simulink model "Shaddad_System"  (R2026b)
undefined symbols (not defined in the file): P, scn_ic_elec_hw, Ts, VC_IMPL
libraries: simulink x4, sl3dlib x1
settings Model: Creator=aomar  LastModifiedBy=aomar

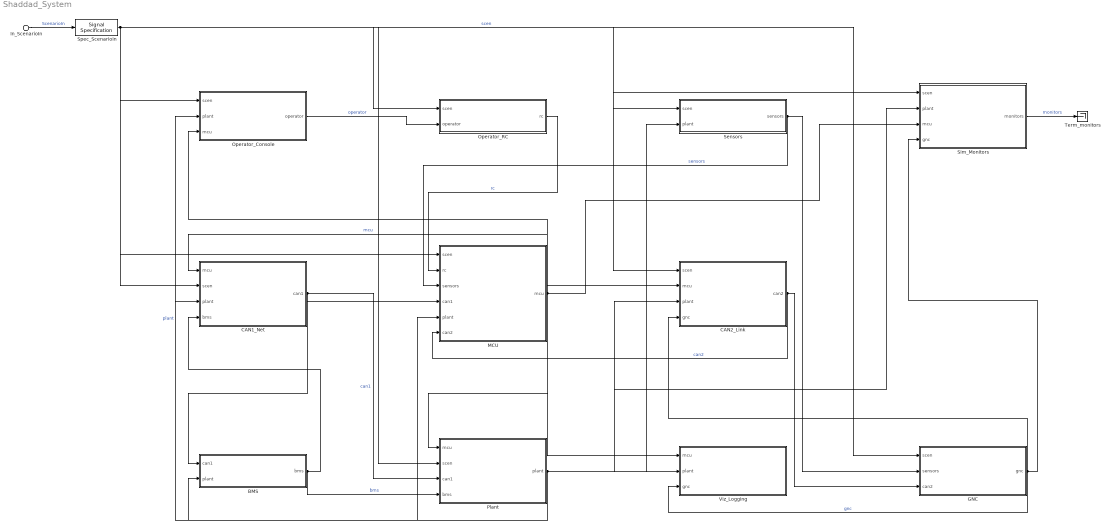
== system Shaddad_System ==
  In_ScenarioIn : Inport  PortName=ScenarioIn
  BMS : Subsystem  Description=BMS (ICD 3.1): Model Shaddad_BMS; its command leaves through BMS_Cmd_Delay (the ECU's one-sample compute delay, rule 8, D36) as bms.cmd_d.
  CAN1_Net : Subsystem
  CAN2_Link : Subsystem
  GNC : Subsystem  Description=GNC (ICD 3.1): MissionCmd_RT (0.01 -> 0.2 s, D32) and GNC_Variant (VC_PHASE 1 GNC_Stub, 2 Model Shaddad_Companion, D38).
  MCU : Subsystem  Description=MCU (ICD 3.1): MCU_In -> Model Shaddad_MCU. The CAN1 feedback frames and the ADC result reach the MCU one sample late (EscFb/EscSlow/Impl/Bms/Adc_Delay, rule 8, D36).
  Operator_Console : Subsystem  Description=VC_OPSRC 1 = ScenarioIn.op, 2 = dashboard (simulink_hmi_blocks bound to Constants, interactive runs), 3 = transmitter in USB joystick mode (Simulation 3D Joystick + joy_map, P.scen.joy), 4 = RC row test driver (row_driver_step, P.scen.rowdrv; fed the delayed true pose, speed, MCU mode and sprayer tank volume).
  Operator_RC : Subsystem
  Plant : Subsystem  Description=Plant (ICD 3.1): Model Shaddad_Plant; the DI word leaves through ElecHw_Delay (sampled by the MCU, rule 8, D36) as plant.elec_hw_d.
  Sensors : Subsystem
  Sim_Monitors : Subsystem
  Spec_ScenarioIn : SignalSpecification  OutDataTypeStr=Bus: Bus_ScenarioIn  SampleTime=Ts.scen  BusOutputAsStruct=on
  Term_monitors : Terminator
  Viz_Logging : Subsystem
  wires:
  In_ScenarioIn/1 -> Spec_ScenarioIn/1  "ScenarioIn"
  Spec_ScenarioIn/1 -> Plant/2(scen), GNC/1(scen), CAN1_Net/2(scen), CAN2_Link/1(scen), MCU/1(scen), Operator_RC/1(scen), Sensors/1(scen), Operator_Console/1(scen), Sim_Monitors/1(scen)  "scen"
  Operator_Console/1(operator) -> Operator_RC/2(operator)  "operator"
  CAN1_Net/1(can1) -> Plant/3(can1), BMS/1(can1), MCU/4(can1)  "can1"
  BMS/1(bms) -> CAN1_Net/4(bms), Plant/4(bms)  "bms"
  Operator_RC/1(rc) -> MCU/2(rc)  "rc"
  MCU/1(mcu) -> Sim_Monitors/3(mcu), Operator_Console/3(mcu), Viz_Logging/1(mcu), Plant/1(mcu), CAN1_Net/1(mcu), CAN2_Link/2(mcu)  "mcu"
  Plant/1(plant) -> Sim_Monitors/2(plant), Operator_Console/2(plant), Sensors/2(plant), CAN1_Net/3(plant), CAN2_Link/3(plant), MCU/5(plant), BMS/2(plant), Viz_Logging/2(plant)  "plant"
  Sensors/1(sensors) -> GNC/2(sensors), MCU/3(sensors)  "sensors"
  CAN2_Link/1(can2) -> GNC/3(can2), MCU/6(can2)  "can2"
  Sim_Monitors/1(monitors) -> Term_monitors/1  "monitors"
  GNC/1(gnc) -> Sim_Monitors/4(gnc), CAN2_Link/4(gnc), Viz_Logging/3(gnc)  "gnc"

== system Shaddad_System/BMS ==
  can1_mcu_slow_rx : Inport  PortName=can1  Element=mcu_slow_rx
  plant_bms_meas : Inport  Port=2  PortName=plant  Element=bms_meas
  BMS_Cmd_Delay : UnitDelay  InitialCondition=P.ic.Bus_BMS_Cmd  SampleTime=Ts.ctrl
  Shaddad_BMS : ModelReference  ModelNameDialog=Shaddad_BMS  SimulationMode=Normal  ModelReferenceVersion=1.1
  Spec_BMS_can_rx : SignalSpecification  OutDataTypeStr=Bus: Bus_Can1_McuSlow  SampleTime=Ts.comm  BusOutputAsStruct=on
  Spec_BMS_meas : SignalSpecification  OutDataTypeStr=Bus: Bus_BMS_Meas  SampleTime=Ts.ctrl  BusOutputAsStruct=on
  bms_cmd_d : Outport  PortName=bms  Element=cmd_d
  bms_can_tx : Outport  PortName=bms  Element=can_tx
  bms_telem : Outport  PortName=bms  Element=telem
  wires:
  plant_bms_meas/1 -> Spec_BMS_meas/1  "bms_meas"
  can1_mcu_slow_rx/1 -> Spec_BMS_can_rx/1  "mcu_slow_rx"
  Spec_BMS_meas/1 -> Shaddad_BMS/1  "meas"
  Spec_BMS_can_rx/1 -> Shaddad_BMS/2  "can_rx"
  Shaddad_BMS/1 -> BMS_Cmd_Delay/1  "cmd"
  Shaddad_BMS/2 -> bms_can_tx/1  "can_tx"
  Shaddad_BMS/3 -> bms_telem/1  "telem"
  BMS_Cmd_Delay/1 -> bms_cmd_d/1  "cmd_d"

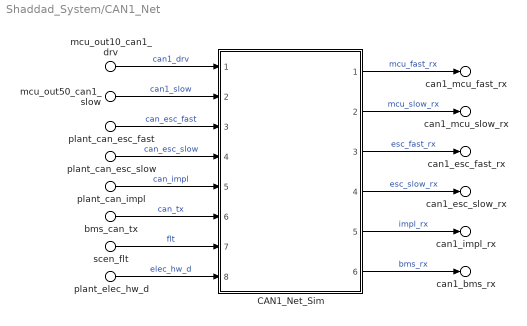
== system Shaddad_System/CAN1_Net ==
  mcu_out10_can1_drv : Inport  PortName=mcu  Element=out10.can1_drv
  mcu_out50_can1_slow : Inport  PortName=mcu  Element=out50.can1_slow
  scen_flt : Inport  Port=2  PortName=scen  Element=flt
  plant_can_esc_fast : Inport  Port=3  PortName=plant  Element=can_esc_fast
  plant_can_esc_slow : Inport  Port=3  PortName=plant  Element=can_esc_slow
  plant_can_impl : Inport  Port=3  PortName=plant  Element=can_impl
  plant_elec_hw_d : Inport  Port=3  PortName=plant  Element=elec_hw_d
  bms_can_tx : Inport  Port=4  PortName=bms  Element=can_tx
  CAN1_Net_Sim : Subsystem  ReferencedSubsystem=CAN1_Net_Sim
  can1_mcu_fast_rx : Outport  PortName=can1  Element=mcu_fast_rx
  can1_mcu_slow_rx : Outport  PortName=can1  Element=mcu_slow_rx
  can1_esc_fast_rx : Outport  PortName=can1  Element=esc_fast_rx
  can1_esc_slow_rx : Outport  PortName=can1  Element=esc_slow_rx
  can1_impl_rx : Outport  PortName=can1  Element=impl_rx
  can1_bms_rx : Outport  PortName=can1  Element=bms_rx
  wires:
  mcu_out10_can1_drv/1 -> CAN1_Net_Sim/1  "can1_drv"
  mcu_out50_can1_slow/1 -> CAN1_Net_Sim/2  "can1_slow"
  plant_can_esc_fast/1 -> CAN1_Net_Sim/3  "can_esc_fast"
  plant_can_esc_slow/1 -> CAN1_Net_Sim/4  "can_esc_slow"
  plant_can_impl/1 -> CAN1_Net_Sim/5  "can_impl"
  bms_can_tx/1 -> CAN1_Net_Sim/6  "can_tx"
  scen_flt/1 -> CAN1_Net_Sim/7  "flt"
  plant_elec_hw_d/1 -> CAN1_Net_Sim/8  "elec_hw_d"
  CAN1_Net_Sim/1 -> can1_mcu_fast_rx/1  "mcu_fast_rx"
  CAN1_Net_Sim/2 -> can1_mcu_slow_rx/1  "mcu_slow_rx"
  CAN1_Net_Sim/3 -> can1_esc_fast_rx/1  "esc_fast_rx"
  CAN1_Net_Sim/4 -> can1_esc_slow_rx/1  "esc_slow_rx"
  CAN1_Net_Sim/5 -> can1_impl_rx/1  "impl_rx"
  CAN1_Net_Sim/6 -> can1_bms_rx/1  "bms_rx"

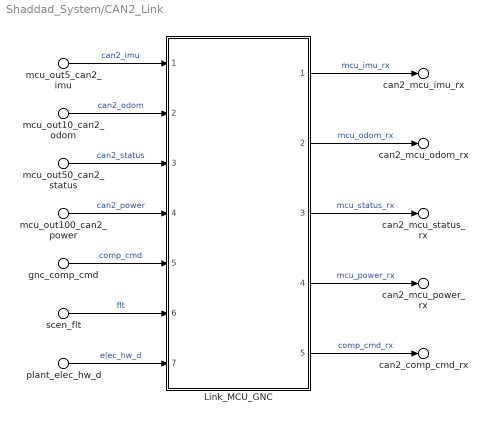
== system Shaddad_System/CAN2_Link ==
  scen_flt : Inport  PortName=scen  Element=flt
  mcu_out5_can2_imu : Inport  Port=2  PortName=mcu  Element=out5.can2_imu
  mcu_out10_can2_odom : Inport  Port=2  PortName=mcu  Element=out10.can2_odom
  mcu_out50_can2_status : Inport  Port=2  PortName=mcu  Element=out50.can2_status
  mcu_out100_can2_power : Inport  Port=2  PortName=mcu  Element=out100.can2_power
  plant_elec_hw_d : Inport  Port=3  PortName=plant  Element=elec_hw_d
  gnc_comp_cmd : Inport  Port=4  PortName=gnc  Element=comp_cmd
  Link_MCU_GNC : Subsystem  ReferencedSubsystem=Link_MCU_GNC
  can2_mcu_imu_rx : Outport  PortName=can2  Element=mcu_imu_rx
  can2_mcu_odom_rx : Outport  PortName=can2  Element=mcu_odom_rx
  can2_mcu_status_rx : Outport  PortName=can2  Element=mcu_status_rx
  can2_mcu_power_rx : Outport  PortName=can2  Element=mcu_power_rx
  can2_comp_cmd_rx : Outport  PortName=can2  Element=comp_cmd_rx
  wires:
  mcu_out5_can2_imu/1 -> Link_MCU_GNC/1  "can2_imu"
  mcu_out10_can2_odom/1 -> Link_MCU_GNC/2  "can2_odom"
  mcu_out50_can2_status/1 -> Link_MCU_GNC/3  "can2_status"
  mcu_out100_can2_power/1 -> Link_MCU_GNC/4  "can2_power"
  gnc_comp_cmd/1 -> Link_MCU_GNC/5  "comp_cmd"
  scen_flt/1 -> Link_MCU_GNC/6  "flt"
  plant_elec_hw_d/1 -> Link_MCU_GNC/7  "elec_hw_d"
  Link_MCU_GNC/1 -> can2_mcu_imu_rx/1  "mcu_imu_rx"
  Link_MCU_GNC/2 -> can2_mcu_odom_rx/1  "mcu_odom_rx"
  Link_MCU_GNC/3 -> can2_mcu_status_rx/1  "mcu_status_rx"
  Link_MCU_GNC/4 -> can2_mcu_power_rx/1  "mcu_power_rx"
  Link_MCU_GNC/5 -> can2_comp_cmd_rx/1  "comp_cmd_rx"

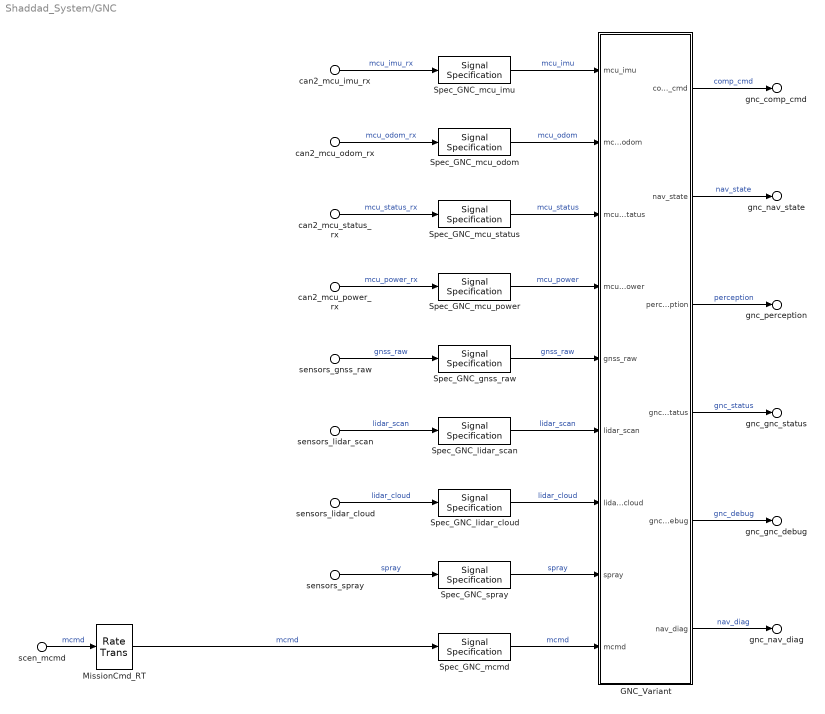
== system Shaddad_System/GNC ==
  scen_mcmd : Inport  PortName=scen  Element=mcmd
  sensors_gnss_raw : Inport  Port=2  PortName=sensors  Element=gnss_raw
  sensors_lidar_scan : Inport  Port=2  PortName=sensors  Element=lidar_scan
  sensors_lidar_cloud : Inport  Port=2  PortName=sensors  Element=lidar_cloud
  sensors_spray : Inport  Port=2  PortName=sensors  Element=spray
  can2_mcu_imu_rx : Inport  Port=3  PortName=can2  Element=mcu_imu_rx
  can2_mcu_odom_rx : Inport  Port=3  PortName=can2  Element=mcu_odom_rx
  can2_mcu_status_rx : Inport  Port=3  PortName=can2  Element=mcu_status_rx
  can2_mcu_power_rx : Inport  Port=3  PortName=can2  Element=mcu_power_rx
  GNC_Variant : Subsystem  Variant=on
  MissionCmd_RT : RateTransition  InitialCondition=P.ic.Bus_MissionCmd  OutPortSampleTime=Ts.mcmd
  Spec_GNC_gnss_raw : SignalSpecification  OutDataTypeStr=Bus: Bus_GnssRaw  SampleTime=Ts.hk  BusOutputAsStruct=on
  Spec_GNC_lidar_cloud : SignalSpecification  OutDataTypeStr=Bus: Bus_LidarCloudRaw  SampleTime=Ts.hk  BusOutputAsStruct=on
  Spec_GNC_lidar_scan : SignalSpecification  OutDataTypeStr=Bus: Bus_LidarScanRaw  SampleTime=Ts.hk  BusOutputAsStruct=on
  Spec_GNC_mcmd : SignalSpecification  OutDataTypeStr=Bus: Bus_MissionCmd  SampleTime=Ts.gnc_status  BusOutputAsStruct=on
  Spec_GNC_mcu_imu : SignalSpecification  OutDataTypeStr=Bus: Bus_CanFrame64  SampleTime=Ts.imu  BusOutputAsStruct=on
  Spec_GNC_mcu_odom : SignalSpecification  OutDataTypeStr=Bus: Bus_CanFrame64  SampleTime=Ts.ctrl  BusOutputAsStruct=on
  Spec_GNC_mcu_power : SignalSpecification  OutDataTypeStr=Bus: Bus_CanFrame64  SampleTime=Ts.hk  BusOutputAsStruct=on
  Spec_GNC_mcu_status : SignalSpecification  OutDataTypeStr=Bus: Bus_CanFrame64  SampleTime=Ts.comm  BusOutputAsStruct=on
  Spec_GNC_spray : SignalSpecification  OutDataTypeStr=Bus: Bus_SprayDemand  SampleTime=Ts.hk  BusOutputAsStruct=on
  gnc_comp_cmd : Outport  PortName=gnc  Element=comp_cmd
  gnc_nav_state : Outport  PortName=gnc  Element=nav_state
  gnc_perception : Outport  PortName=gnc  Element=perception
  gnc_gnc_status : Outport  PortName=gnc  Element=gnc_status
  gnc_gnc_debug : Outport  PortName=gnc  Element=gnc_debug
  gnc_nav_diag : Outport  PortName=gnc  Element=nav_diag
  wires:
  scen_mcmd/1 -> MissionCmd_RT/1  "mcmd"
  MissionCmd_RT/1 -> Spec_GNC_mcmd/1  "mcmd"
  can2_mcu_imu_rx/1 -> Spec_GNC_mcu_imu/1  "mcu_imu_rx"
  can2_mcu_odom_rx/1 -> Spec_GNC_mcu_odom/1  "mcu_odom_rx"
  can2_mcu_status_rx/1 -> Spec_GNC_mcu_status/1  "mcu_status_rx"
  can2_mcu_power_rx/1 -> Spec_GNC_mcu_power/1  "mcu_power_rx"
  sensors_gnss_raw/1 -> Spec_GNC_gnss_raw/1  "gnss_raw"
  sensors_lidar_scan/1 -> Spec_GNC_lidar_scan/1  "lidar_scan"
  sensors_lidar_cloud/1 -> Spec_GNC_lidar_cloud/1  "lidar_cloud"
  sensors_spray/1 -> Spec_GNC_spray/1  "spray"
  Spec_GNC_mcu_imu/1 -> GNC_Variant/1(mcu_imu)  "mcu_imu"
  Spec_GNC_mcu_odom/1 -> GNC_Variant/2(mcu_odom)  "mcu_odom"
  Spec_GNC_mcu_status/1 -> GNC_Variant/3(mcu_status)  "mcu_status"
  Spec_GNC_mcu_power/1 -> GNC_Variant/4(mcu_power)  "mcu_power"
  Spec_GNC_gnss_raw/1 -> GNC_Variant/5(gnss_raw)  "gnss_raw"
  Spec_GNC_lidar_scan/1 -> GNC_Variant/6(lidar_scan)  "lidar_scan"
  Spec_GNC_lidar_cloud/1 -> GNC_Variant/7(lidar_cloud)  "lidar_cloud"
  Spec_GNC_spray/1 -> GNC_Variant/8(spray)  "spray"
  Spec_GNC_mcmd/1 -> GNC_Variant/9(mcmd)  "mcmd"
  GNC_Variant/1(comp_cmd) -> gnc_comp_cmd/1  "comp_cmd"
  GNC_Variant/2(nav_state) -> gnc_nav_state/1  "nav_state"
  GNC_Variant/3(perception) -> gnc_perception/1  "perception"
  GNC_Variant/4(gnc_status) -> gnc_gnc_status/1  "gnc_status"
  GNC_Variant/5(gnc_debug) -> gnc_gnc_debug/1  "gnc_debug"
  GNC_Variant/6(nav_diag) -> gnc_nav_diag/1  "nav_diag"

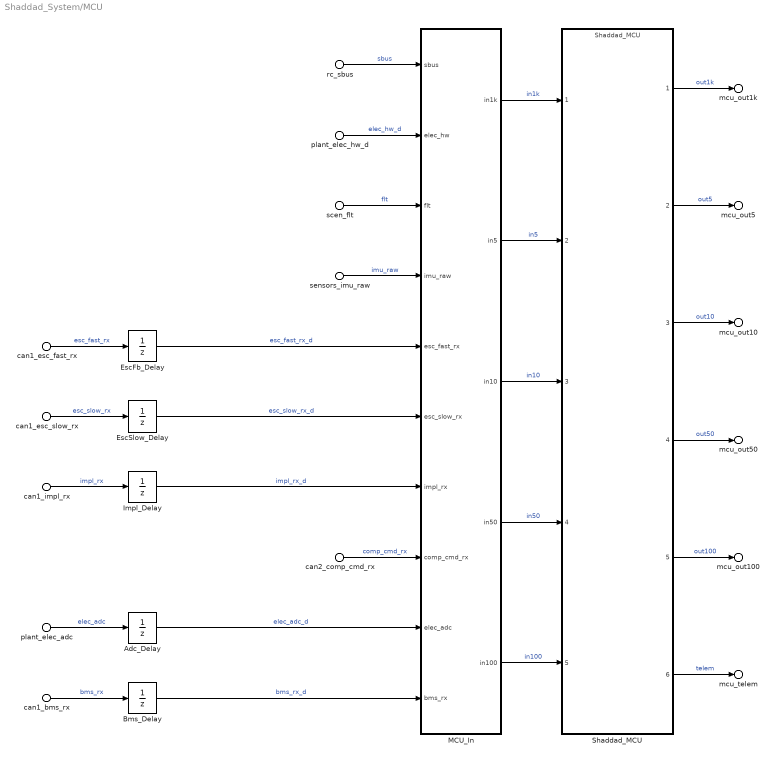
== system Shaddad_System/MCU ==
  scen_flt : Inport  PortName=scen  Element=flt
  rc_sbus : Inport  Port=2  PortName=rc  Element=sbus
  sensors_imu_raw : Inport  Port=3  PortName=sensors  Element=imu_raw
  can1_esc_fast_rx : Inport  Port=4  PortName=can1  Element=esc_fast_rx
  can1_esc_slow_rx : Inport  Port=4  PortName=can1  Element=esc_slow_rx
  can1_impl_rx : Inport  Port=4  PortName=can1  Element=impl_rx
  can1_bms_rx : Inport  Port=4  PortName=can1  Element=bms_rx
  plant_elec_hw_d : Inport  Port=5  PortName=plant  Element=elec_hw_d
  plant_elec_adc : Inport  Port=5  PortName=plant  Element=elec_adc
  can2_comp_cmd_rx : Inport  Port=6  PortName=can2  Element=comp_cmd_rx
  Adc_Delay : UnitDelay  InitialCondition=P.ic.Bus_ElecAdc  SampleTime=Ts.comm
  Bms_Delay : UnitDelay  InitialCondition=P.ic.Bus_Can1_Bms  SampleTime=Ts.hk
  EscFb_Delay : UnitDelay  InitialCondition=P.ic.Bus_Can1_EscFast  SampleTime=Ts.ctrl
  EscSlow_Delay : UnitDelay  InitialCondition=P.ic.Bus_Can1_EscSlow  SampleTime=Ts.comm
  Impl_Delay : UnitDelay  InitialCondition=P.ic.Bus_Can1_Impl  SampleTime=Ts.comm
  MCU_In : Subsystem  Description=MCU input assembly: explicit deterministic Rate Transitions to the task rates, nonvirtual Bus_McuIn* Bus Creators, t_us (1 MHz, wraps 2^32) and the SIM fault_inject word (ICD 6).
  Shaddad_MCU : ModelReference  ModelNameDialog=Shaddad_MCU  SimulationMode=Normal  ModelReferenceVersion=1.1
  mcu_out1k : Outport  PortName=mcu  Element=out1k
  mcu_out5 : Outport  PortName=mcu  Element=out5
  mcu_out10 : Outport  PortName=mcu  Element=out10
  mcu_out50 : Outport  PortName=mcu  Element=out50
  mcu_out100 : Outport  PortName=mcu  Element=out100
  mcu_telem : Outport  PortName=mcu  Element=telem
  wires:
  can1_esc_fast_rx/1 -> EscFb_Delay/1  "esc_fast_rx"
  can1_esc_slow_rx/1 -> EscSlow_Delay/1  "esc_slow_rx"
  can1_impl_rx/1 -> Impl_Delay/1  "impl_rx"
  plant_elec_adc/1 -> Adc_Delay/1  "elec_adc"
  can1_bms_rx/1 -> Bms_Delay/1  "bms_rx"
  EscFb_Delay/1 -> MCU_In/5(esc_fast_rx)  "esc_fast_rx_d"
  EscSlow_Delay/1 -> MCU_In/6(esc_slow_rx)  "esc_slow_rx_d"
  Impl_Delay/1 -> MCU_In/7(impl_rx)  "impl_rx_d"
  Adc_Delay/1 -> MCU_In/9(elec_adc)  "elec_adc_d"
  Bms_Delay/1 -> MCU_In/10(bms_rx)  "bms_rx_d"
  rc_sbus/1 -> MCU_In/1(sbus)  "sbus"
  plant_elec_hw_d/1 -> MCU_In/2(elec_hw)  "elec_hw_d"
  scen_flt/1 -> MCU_In/3(flt)  "flt"
  sensors_imu_raw/1 -> MCU_In/4(imu_raw)  "imu_raw"
  can2_comp_cmd_rx/1 -> MCU_In/8(comp_cmd_rx)  "comp_cmd_rx"
  MCU_In/1(in1k) -> Shaddad_MCU/1  "in1k"
  MCU_In/2(in5) -> Shaddad_MCU/2  "in5"
  MCU_In/3(in10) -> Shaddad_MCU/3  "in10"
  MCU_In/4(in50) -> Shaddad_MCU/4  "in50"
  MCU_In/5(in100) -> Shaddad_MCU/5  "in100"
  Shaddad_MCU/1 -> mcu_out1k/1  "out1k"
  Shaddad_MCU/2 -> mcu_out5/1  "out5"
  Shaddad_MCU/3 -> mcu_out10/1  "out10"
  Shaddad_MCU/4 -> mcu_out50/1  "out50"
  Shaddad_MCU/5 -> mcu_out100/1  "out100"
  Shaddad_MCU/6 -> mcu_telem/1  "telem"

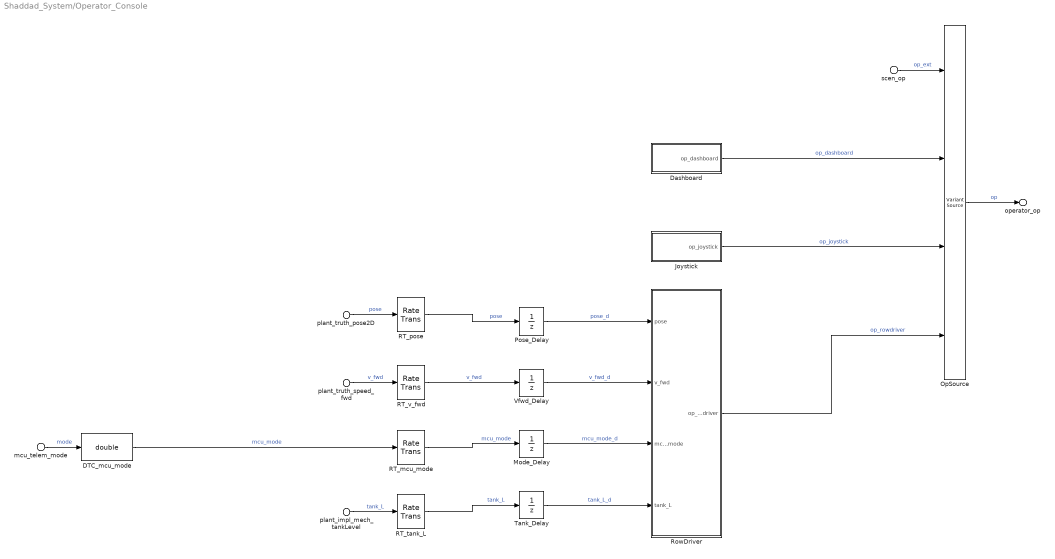
== system Shaddad_System/Operator_Console ==
  scen_op : Inport  PortName=scen  Element=op
  plant_truth_pose2D : Inport  Port=2  PortName=plant  Element=truth.pose2D
  plant_truth_speed_fwd : Inport  Port=2  PortName=plant  Element=truth.speed_fwd
  plant_impl_mech_tankLevel : Inport  Port=2  PortName=plant  Element=impl_mech.tankLevel
  mcu_telem_mode : Inport  Port=3  PortName=mcu  Element=telem.mode
  DTC_mcu_mode : DataTypeConversion  OutDataTypeStr=double  SaturateOnIntegerOverflow=off  RndMeth=Floor
  Dashboard : Subsystem  Description=VC_OPSRC 2: dashboard RC (simulink_hmi_blocks bound to the P.scen.dash Constants).
  Joystick : Subsystem  Description=VC_OPSRC 3: real transmitter in USB joystick mode (Simulation 3D Joystick, ID 1) mapped by utilities/joy_map.m with P.scen.joy; run phase1_live_drive('Source','joystick').
  Mode_Delay : UnitDelay  SampleTime=Ts.scen
  OpSource : VariantSource  VariantControls={VC_OPSRC == 1, VC_OPSRC == 2, VC_OPSRC == 3, VC_OPSRC == 4}
  Pose_Delay : UnitDelay  InitialCondition=P.structure.init.pose2D0  SampleTime=Ts.scen
  RT_mcu_mode : RateTransition  OutPortSampleTime=Ts.scen
  RT_pose : RateTransition  InitialCondition=P.structure.init.pose2D0  OutPortSampleTime=Ts.scen
  RT_tank_L : RateTransition  OutPortSampleTime=Ts.scen
  RT_v_fwd : RateTransition  OutPortSampleTime=Ts.scen
  RowDriver : Subsystem  Description=VC_OPSRC 4: RC row test driver (scenario R1, phase1_row_test): delayed true pose / speed, MCU mode and sprayer tank volume -> sticks and switches (the pump off once the tank is empty); Stop Simulation once the driver has ended the run.
  Tank_Delay : UnitDelay  SampleTime=Ts.scen
  Vfwd_Delay : UnitDelay  SampleTime=Ts.scen
  operator_op : Outport  PortName=operator  Element=op
  wires:
  mcu_telem_mode/1 -> DTC_mcu_mode/1  "mode"
  DTC_mcu_mode/1 -> RT_mcu_mode/1  "mcu_mode"
  plant_truth_pose2D/1 -> RT_pose/1  "pose"
  plant_truth_speed_fwd/1 -> RT_v_fwd/1  "v_fwd"
  plant_impl_mech_tankLevel/1 -> RT_tank_L/1  "tank_L"
  RT_pose/1 -> Pose_Delay/1  "pose"
  RT_v_fwd/1 -> Vfwd_Delay/1  "v_fwd"
  RT_mcu_mode/1 -> Mode_Delay/1  "mcu_mode"
  RT_tank_L/1 -> Tank_Delay/1  "tank_L"
  Pose_Delay/1 -> RowDriver/1(pose)  "pose_d"
  Vfwd_Delay/1 -> RowDriver/2(v_fwd)  "v_fwd_d"
  Mode_Delay/1 -> RowDriver/3(mcu_mode)  "mcu_mode_d"
  Tank_Delay/1 -> RowDriver/4(tank_L)  "tank_L_d"
  Dashboard/1(op_dashboard) -> OpSource/2  "op_dashboard"
  Joystick/1(op_joystick) -> OpSource/3  "op_joystick"
  RowDriver/1(op_rowdriver) -> OpSource/4  "op_rowdriver"
  scen_op/1 -> OpSource/1  "op_ext"
  OpSource/1 -> operator_op/1  "op"

== system Shaddad_System/Operator_RC ==
  scen_flt : Inport  PortName=scen  Element=flt
  operator_op : Inport  Port=2  PortName=operator  Element=op
  RC_Link_Sim : Subsystem  ReferencedSubsystem=RC_Link_Sim
  rc_sbus : Outport  PortName=rc  Element=sbus
  rc_rc_frame : Outport  PortName=rc  Element=rc_frame
  wires:
  operator_op/1 -> RC_Link_Sim/1  "op"
  scen_flt/1 -> RC_Link_Sim/2  "flt"
  RC_Link_Sim/1 -> rc_sbus/1  "sbus"
  RC_Link_Sim/2 -> rc_rc_frame/1  "rc_frame"

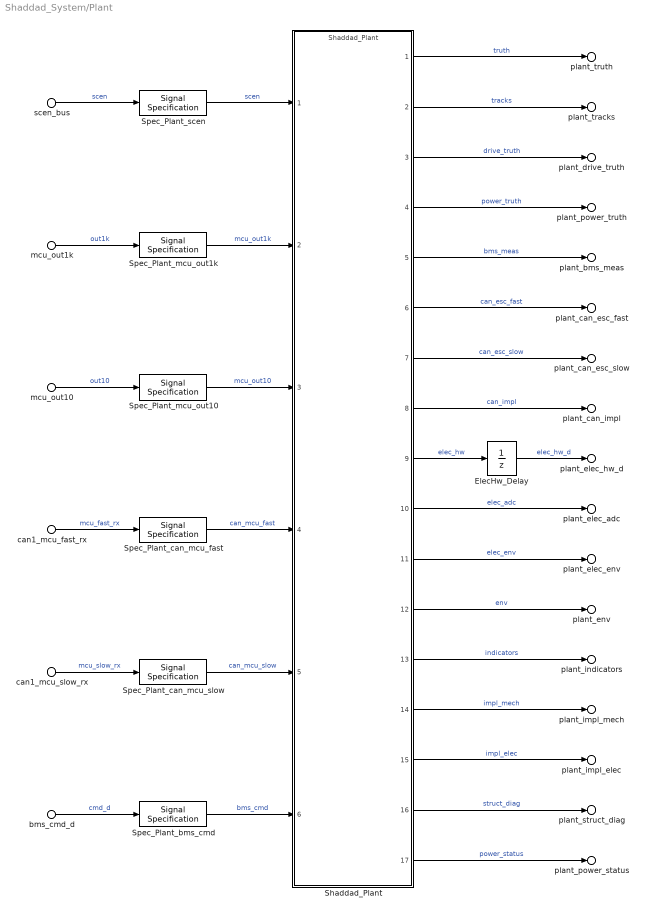
== system Shaddad_System/Plant ==
  mcu_out1k : Inport  PortName=mcu  Element=out1k
  mcu_out10 : Inport  PortName=mcu  Element=out10
  scen_bus : Inport  Port=2  PortName=scen
  can1_mcu_fast_rx : Inport  Port=3  PortName=can1  Element=mcu_fast_rx
  can1_mcu_slow_rx : Inport  Port=3  PortName=can1  Element=mcu_slow_rx
  bms_cmd_d : Inport  Port=4  PortName=bms  Element=cmd_d
  ElecHw_Delay : UnitDelay  InitialCondition=scn_ic_elec_hw(P, VC_IMPL)  SampleTime=Ts.base
  Shaddad_Plant : ModelReference  ModelNameDialog=Shaddad_Plant  SimulationMode=Normal  ModelReferenceVersion=1.1
  Spec_Plant_bms_cmd : SignalSpecification  OutDataTypeStr=Bus: Bus_BMS_Cmd  SampleTime=Ts.ctrl  BusOutputAsStruct=on
  Spec_Plant_can_mcu_fast : SignalSpecification  OutDataTypeStr=Bus: Bus_Can1_McuFast  SampleTime=Ts.ctrl  BusOutputAsStruct=on
  Spec_Plant_can_mcu_slow : SignalSpecification  OutDataTypeStr=Bus: Bus_Can1_McuSlow  SampleTime=Ts.comm  BusOutputAsStruct=on
  Spec_Plant_mcu_out10 : SignalSpecification  OutDataTypeStr=Bus: Bus_McuOut10  SampleTime=Ts.ctrl  BusOutputAsStruct=on
  Spec_Plant_mcu_out1k : SignalSpecification  OutDataTypeStr=Bus: Bus_McuOut1k  SampleTime=Ts.base  BusOutputAsStruct=on
  Spec_Plant_scen : SignalSpecification  OutDataTypeStr=Bus: Bus_ScenarioIn  SampleTime=Ts.ctrl  BusOutputAsStruct=on
  plant_truth : Outport  PortName=plant  Element=truth
  plant_tracks : Outport  PortName=plant  Element=tracks
  plant_drive_truth : Outport  PortName=plant  Element=drive_truth
  plant_power_truth : Outport  PortName=plant  Element=power_truth
  plant_bms_meas : Outport  PortName=plant  Element=bms_meas
  plant_can_esc_fast : Outport  PortName=plant  Element=can_esc_fast
  plant_can_esc_slow : Outport  PortName=plant  Element=can_esc_slow
  plant_can_impl : Outport  PortName=plant  Element=can_impl
  plant_elec_hw_d : Outport  PortName=plant  Element=elec_hw_d
  plant_elec_adc : Outport  PortName=plant  Element=elec_adc
  plant_elec_env : Outport  PortName=plant  Element=elec_env
  plant_env : Outport  PortName=plant  Element=env
  plant_indicators : Outport  PortName=plant  Element=indicators
  plant_impl_mech : Outport  PortName=plant  Element=impl_mech
  plant_impl_elec : Outport  PortName=plant  Element=impl_elec
  plant_struct_diag : Outport  PortName=plant  Element=struct_diag
  plant_power_status : Outport  PortName=plant  Element=power_status
  wires:
  scen_bus/1 -> Spec_Plant_scen/1  "scen"
  mcu_out1k/1 -> Spec_Plant_mcu_out1k/1  "out1k"
  mcu_out10/1 -> Spec_Plant_mcu_out10/1  "out10"
  can1_mcu_fast_rx/1 -> Spec_Plant_can_mcu_fast/1  "mcu_fast_rx"
  can1_mcu_slow_rx/1 -> Spec_Plant_can_mcu_slow/1  "mcu_slow_rx"
  bms_cmd_d/1 -> Spec_Plant_bms_cmd/1  "cmd_d"
  Spec_Plant_scen/1 -> Shaddad_Plant/1  "scen"
  Spec_Plant_mcu_out1k/1 -> Shaddad_Plant/2  "mcu_out1k"
  Spec_Plant_mcu_out10/1 -> Shaddad_Plant/3  "mcu_out10"
  Spec_Plant_can_mcu_fast/1 -> Shaddad_Plant/4  "can_mcu_fast"
  Spec_Plant_can_mcu_slow/1 -> Shaddad_Plant/5  "can_mcu_slow"
  Spec_Plant_bms_cmd/1 -> Shaddad_Plant/6  "bms_cmd"
  Shaddad_Plant/1 -> plant_truth/1  "truth"
  Shaddad_Plant/2 -> plant_tracks/1  "tracks"
  Shaddad_Plant/3 -> plant_drive_truth/1  "drive_truth"
  Shaddad_Plant/4 -> plant_power_truth/1  "power_truth"
  Shaddad_Plant/5 -> plant_bms_meas/1  "bms_meas"
  Shaddad_Plant/6 -> plant_can_esc_fast/1  "can_esc_fast"
  Shaddad_Plant/7 -> plant_can_esc_slow/1  "can_esc_slow"
  Shaddad_Plant/8 -> plant_can_impl/1  "can_impl"
  Shaddad_Plant/9 -> ElecHw_Delay/1  "elec_hw"
  Shaddad_Plant/10 -> plant_elec_adc/1  "elec_adc"
  Shaddad_Plant/11 -> plant_elec_env/1  "elec_env"
  Shaddad_Plant/12 -> plant_env/1  "env"
  Shaddad_Plant/13 -> plant_indicators/1  "indicators"
  Shaddad_Plant/14 -> plant_impl_mech/1  "impl_mech"
  Shaddad_Plant/15 -> plant_impl_elec/1  "impl_elec"
  Shaddad_Plant/16 -> plant_struct_diag/1  "struct_diag"
  Shaddad_Plant/17 -> plant_power_status/1  "power_status"
  ElecHw_Delay/1 -> plant_elec_hw_d/1  "elec_hw_d"

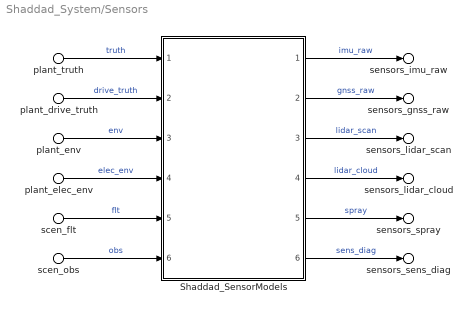
== system Shaddad_System/Sensors ==
  scen_flt : Inport  PortName=scen  Element=flt
  scen_obs : Inport  PortName=scen  Element=obs
  plant_truth : Inport  Port=2  PortName=plant  Element=truth
  plant_drive_truth : Inport  Port=2  PortName=plant  Element=drive_truth
  plant_env : Inport  Port=2  PortName=plant  Element=env
  plant_elec_env : Inport  Port=2  PortName=plant  Element=elec_env
  Shaddad_SensorModels : Subsystem  ReferencedSubsystem=Shaddad_SensorModels
  sensors_imu_raw : Outport  PortName=sensors  Element=imu_raw
  sensors_gnss_raw : Outport  PortName=sensors  Element=gnss_raw
  sensors_lidar_scan : Outport  PortName=sensors  Element=lidar_scan
  sensors_lidar_cloud : Outport  PortName=sensors  Element=lidar_cloud
  sensors_spray : Outport  PortName=sensors  Element=spray
  sensors_sens_diag : Outport  PortName=sensors  Element=sens_diag
  wires:
  plant_truth/1 -> Shaddad_SensorModels/1  "truth"
  plant_drive_truth/1 -> Shaddad_SensorModels/2  "drive_truth"
  plant_env/1 -> Shaddad_SensorModels/3  "env"
  plant_elec_env/1 -> Shaddad_SensorModels/4  "elec_env"
  scen_flt/1 -> Shaddad_SensorModels/5  "flt"
  scen_obs/1 -> Shaddad_SensorModels/6  "obs"
  Shaddad_SensorModels/1 -> sensors_imu_raw/1  "imu_raw"
  Shaddad_SensorModels/2 -> sensors_gnss_raw/1  "gnss_raw"
  Shaddad_SensorModels/3 -> sensors_lidar_scan/1  "lidar_scan"
  Shaddad_SensorModels/4 -> sensors_lidar_cloud/1  "lidar_cloud"
  Shaddad_SensorModels/5 -> sensors_spray/1  "spray"
  Shaddad_SensorModels/6 -> sensors_sens_diag/1  "sens_diag"

== system Shaddad_System/Sim_Monitors ==
  scen_obs : Inport  PortName=scen  Element=obs
  plant_truth : Inport  Port=2  PortName=plant  Element=truth
  plant_power_truth : Inport  Port=2  PortName=plant  Element=power_truth
  plant_drive_truth : Inport  Port=2  PortName=plant  Element=drive_truth
  plant_struct_diag : Inport  Port=2  PortName=plant  Element=struct_diag
  mcu_telem : Inport  Port=3  PortName=mcu  Element=telem
  gnc_gnc_status : Inport  Port=4  PortName=gnc  Element=gnc_status
  Sim_Monitors : Subsystem  ReferencedSubsystem=Sim_Monitors
  monitors_kpi : Outport  PortName=monitors  Element=kpi
  wires:
  plant_truth/1 -> Sim_Monitors/1  "truth"
  plant_power_truth/1 -> Sim_Monitors/2  "power_truth"
  plant_drive_truth/1 -> Sim_Monitors/3  "drive_truth"
  scen_obs/1 -> Sim_Monitors/4  "obs"
  mcu_telem/1 -> Sim_Monitors/5  "telem"
  gnc_gnc_status/1 -> Sim_Monitors/6  "gnc_status"
  plant_struct_diag/1 -> Sim_Monitors/7  "struct_diag"
  Sim_Monitors/1 -> monitors_kpi/1  "kpi"

== system Shaddad_System/Viz_Logging ==
  mcu_telem : Inport  PortName=mcu  Element=telem
  plant_truth : Inport  Port=2  PortName=plant  Element=truth
  plant_indicators : Inport  Port=2  PortName=plant  Element=indicators
  gnc_nav_state : Inport  Port=3  PortName=gnc  Element=nav_state
  gnc_gnc_status : Inport  Port=3  PortName=gnc  Element=gnc_status
  gnc_perception : Inport  Port=3  PortName=gnc  Element=perception
  Viz_Logging : Subsystem  ReferencedSubsystem=Viz_Logging
  wires:
  plant_truth/1 -> Viz_Logging/1  "truth"
  gnc_nav_state/1 -> Viz_Logging/2  "nav_state"
  gnc_gnc_status/1 -> Viz_Logging/3  "gnc_status"
  gnc_perception/1 -> Viz_Logging/4  "perception"
  mcu_telem/1 -> Viz_Logging/5  "telem"
  plant_indicators/1 -> Viz_Logging/6  "indicators"

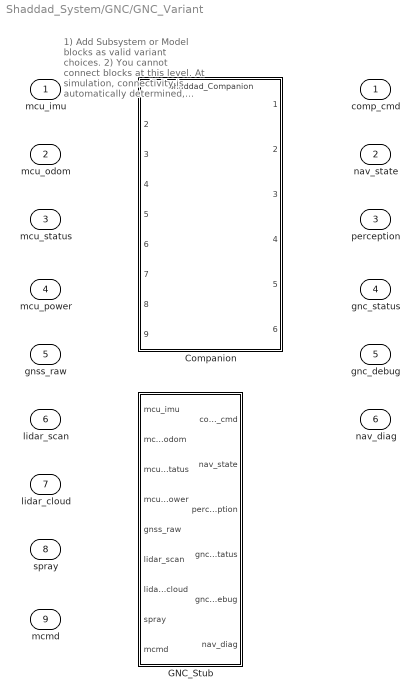
== system Shaddad_System/GNC/GNC_Variant ==
  note: 1) Add Subsystem or Model blocks as valid variant choices.
      | 2) You cannot connect blocks at this level. At simulation, connectivity is automatically
      | determined, based on the active variant and port name matching.
  mcu_imu : Inport
  mcu_odom : Inport  Port=2
  mcu_status : Inport  Port=3
  mcu_power : Inport  Port=4
  gnss_raw : Inport  Port=5
  lidar_scan : Inport  Port=6
  lidar_cloud : Inport  Port=7
  spray : Inport  Port=8
  mcmd : Inport  Port=9
  Companion : ModelReference  ModelNameDialog=Shaddad_Companion  SimulationMode=Normal  VariantControl=VC_PHASE == 2  ModelReferenceVersion=1.1
  GNC_Stub : Subsystem  Description=Phase 1 (RC only): no companion; COMP_CMD valid = false so the MCU never sees comp_ok.  VariantControl=VC_PHASE == 1
  comp_cmd : Outport
  nav_state : Outport  Port=2
  perception : Outport  Port=3
  gnc_status : Outport  Port=4
  gnc_debug : Outport  Port=5
  nav_diag : Outport  Port=6

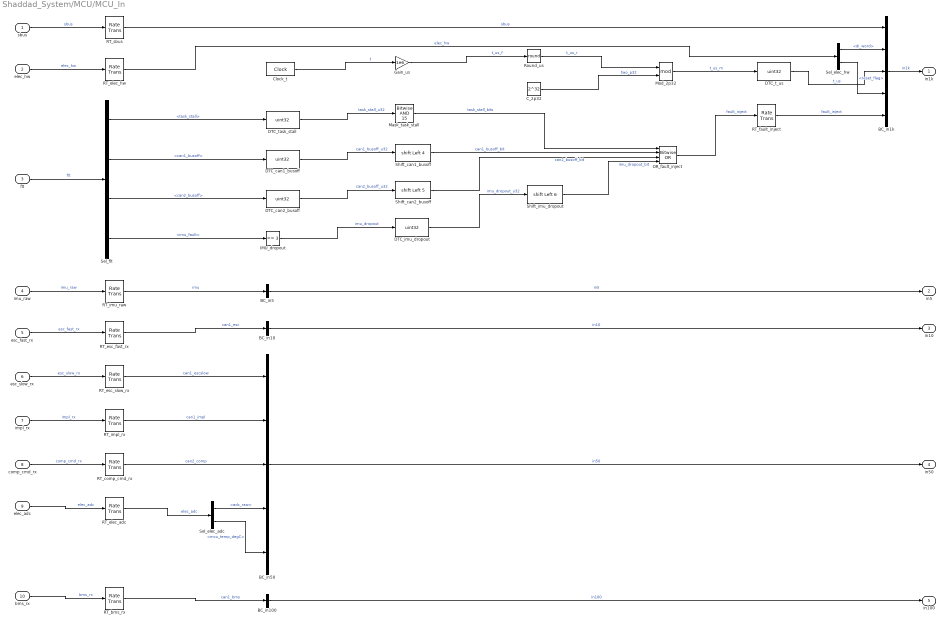
== system Shaddad_System/MCU/MCU_In ==
  sbus : Inport  OutDataTypeStr=Bus: Bus_SbusStream
  elec_hw : Inport  Port=2  OutDataTypeStr=Bus: Bus_ElecHwIn
  flt : Inport  Port=3  OutDataTypeStr=Bus: Bus_FaultInject
  imu_raw : Inport  Port=4  OutDataTypeStr=Bus: Bus_ImuRaw
  esc_fast_rx : Inport  Port=5  OutDataTypeStr=Bus: Bus_Can1_EscFast
  esc_slow_rx : Inport  Port=6  OutDataTypeStr=Bus: Bus_Can1_EscSlow
  impl_rx : Inport  Port=7  OutDataTypeStr=Bus: Bus_Can1_Impl
  comp_cmd_rx : Inport  Port=8  OutDataTypeStr=Bus: Bus_CanFrame64
  elec_adc : Inport  Port=9  OutDataTypeStr=Bus: Bus_ElecAdc
  bms_rx : Inport  Port=10  OutDataTypeStr=Bus: Bus_Can1_Bms
  BC_in10 : BusCreator  Inputs=1  OutDataTypeStr=Bus: Bus_McuIn10  NonVirtualBus=on
  BC_in100 : BusCreator  Inputs=1  OutDataTypeStr=Bus: Bus_McuIn100  NonVirtualBus=on
  BC_in1k : BusCreator  Inputs=5  OutDataTypeStr=Bus: Bus_McuIn1k  NonVirtualBus=on
  BC_in5 : BusCreator  Inputs=1  OutDataTypeStr=Bus: Bus_McuIn5  NonVirtualBus=on
  BC_in50 : BusCreator  Inputs=5  OutDataTypeStr=Bus: Bus_McuIn50  NonVirtualBus=on
  C_2p32 : Constant  Value=2^32
  Clock_t : DigitalClock  SampleTime=Ts.base
  DTC_can1_busoff : DataTypeConversion  OutDataTypeStr=uint32  SaturateOnIntegerOverflow=off  RndMeth=Floor
  DTC_can2_busoff : DataTypeConversion  OutDataTypeStr=uint32  SaturateOnIntegerOverflow=off  RndMeth=Floor
  DTC_imu_dropout : DataTypeConversion  OutDataTypeStr=uint32  SaturateOnIntegerOverflow=off  RndMeth=Floor
  DTC_t_us : DataTypeConversion  OutDataTypeStr=uint32  SaturateOnIntegerOverflow=off  RndMeth=Floor
  DTC_task_stall : DataTypeConversion  OutDataTypeStr=uint32  SaturateOnIntegerOverflow=off  RndMeth=Floor
  Gain_us : Gain  Gain=1e6
  IMU_dropout : simulink/Logic and Bit Operations/Compare To Constant  relop===  const=3  OutDataTypeStr=boolean
  Mask_task_stall : simulink/Logic and Bit Operations/Bitwise Operator  logicop=AND  UseBitMask=on  BitMask=15  BitMaskRealWorld=Stored Integer
  Mod_2p32 : Math  Operator=mod
  OR_fault_inject : simulink/Logic and Bit Operations/Bitwise Operator  logicop=OR  UseBitMask=off  NumInputPorts=4  BitMask=bin2dec('11011001')  BitMaskRealWorld=Stored Integer
  RT_bms_rx : RateTransition  InitialCondition=P.ic.Bus_Can1_Bms  OutPortSampleTime=Ts.hk
  RT_comp_cmd_rx : RateTransition  InitialCondition=P.ic.Bus_CanFrame64  OutPortSampleTime=Ts.comm
  RT_elec_adc : RateTransition  InitialCondition=P.ic.Bus_ElecAdc  OutPortSampleTime=Ts.comm
  RT_elec_hw : RateTransition  InitialCondition=P.ic.Bus_ElecHwIn  OutPortSampleTime=Ts.base
  RT_esc_fast_rx : RateTransition  InitialCondition=P.ic.Bus_Can1_EscFast  OutPortSampleTime=Ts.ctrl
  RT_esc_slow_rx : RateTransition  InitialCondition=P.ic.Bus_Can1_EscSlow  OutPortSampleTime=Ts.comm
  RT_fault_inject : RateTransition  OutPortSampleTime=Ts.base
  RT_impl_rx : RateTransition  InitialCondition=P.ic.Bus_Can1_Impl  OutPortSampleTime=Ts.comm
  RT_imu_raw : RateTransition  InitialCondition=P.ic.Bus_ImuRaw  OutPortSampleTime=Ts.imu
  RT_sbus : RateTransition  InitialCondition=P.ic.Bus_SbusStream  OutPortSampleTime=Ts.base
  Round_us : Rounding  Operator=round
  Sel_elec_adc : BusSelector  OutputSignals=adc_raw,mcu_temp_degC
  Sel_elec_hw : BusSelector  OutputSignals=di_word,reset_flag
  Sel_flt : BusSelector  OutputSignals=task_stall,can1_busoff,can2_busoff,imu_fault
  Shift_can1_busoff : ArithShift  BitShiftNumber=4  BitShiftDirection=Left
  Shift_can2_busoff : ArithShift  BitShiftNumber=5  BitShiftDirection=Left
  Shift_imu_dropout : ArithShift  BitShiftNumber=6  BitShiftDirection=Left
  in1k : Outport  OutDataTypeStr=Bus: Bus_McuIn1k
  in5 : Outport  Port=2  OutDataTypeStr=Bus: Bus_McuIn5
  in10 : Outport  Port=3  OutDataTypeStr=Bus: Bus_McuIn10
  in50 : Outport  Port=4  OutDataTypeStr=Bus: Bus_McuIn50
  in100 : Outport  Port=5  OutDataTypeStr=Bus: Bus_McuIn100
  wires:
  sbus/1 -> RT_sbus/1  "sbus"
  elec_hw/1 -> RT_elec_hw/1  "elec_hw"
  flt/1 -> Sel_flt/1  "flt"
  imu_raw/1 -> RT_imu_raw/1  "imu_raw"
  esc_fast_rx/1 -> RT_esc_fast_rx/1  "esc_fast_rx"
  esc_slow_rx/1 -> RT_esc_slow_rx/1  "esc_slow_rx"
  impl_rx/1 -> RT_impl_rx/1  "impl_rx"
  comp_cmd_rx/1 -> RT_comp_cmd_rx/1  "comp_cmd_rx"
  elec_adc/1 -> RT_elec_adc/1  "elec_adc"
  bms_rx/1 -> RT_bms_rx/1  "bms_rx"
  Sel_flt/1 -> DTC_task_stall/1  "<task_stall>"
  Sel_flt/2 -> DTC_can1_busoff/1  "<can1_busoff>"
  Sel_flt/3 -> DTC_can2_busoff/1  "<can2_busoff>"
  Sel_flt/4 -> IMU_dropout/1  "<imu_fault>"
  RT_sbus/1 -> BC_in1k/1  "sbus"
  RT_elec_hw/1 -> Sel_elec_hw/1  "elec_hw"
  RT_imu_raw/1 -> BC_in5/1  "imu"
  RT_esc_fast_rx/1 -> BC_in10/1  "can1_esc"
  RT_esc_slow_rx/1 -> BC_in50/1  "can1_escslow"
  RT_impl_rx/1 -> BC_in50/2  "can1_impl"
  RT_comp_cmd_rx/1 -> BC_in50/3  "can2_comp"
  RT_elec_adc/1 -> Sel_elec_adc/1  "elec_adc"
  RT_bms_rx/1 -> BC_in100/1  "can1_bms"
  Sel_elec_adc/1 -> BC_in50/4  "<adc_raw>"
  Sel_elec_adc/2 -> BC_in50/5  "<mcu_temp_degC>"
  BC_in5/1 -> in5/1  "in5"
  BC_in10/1 -> in10/1  "in10"
  BC_in50/1 -> in50/1  "in50"
  BC_in100/1 -> in100/1  "in100"
  IMU_dropout/1 -> DTC_imu_dropout/1  "imu_dropout"
  Clock_t/1 -> Gain_us/1  "t"
  DTC_task_stall/1 -> Mask_task_stall/1  "task_stall_u32"
  DTC_can1_busoff/1 -> Shift_can1_busoff/1  "can1_busoff_u32"
  DTC_can2_busoff/1 -> Shift_can2_busoff/1  "can2_busoff_u32"
  Gain_us/1 -> Round_us/1  "t_us_f"
  Mask_task_stall/1 -> OR_fault_inject/1  "task_stall_bits"
  DTC_imu_dropout/1 -> Shift_imu_dropout/1  "imu_dropout_u32"
  Shift_can1_busoff/1 -> OR_fault_inject/2  "can1_busoff_bit"
  Shift_can2_busoff/1 -> OR_fault_inject/3  "can2_busoff_bit"
  Round_us/1 -> Mod_2p32/1  "t_us_r"
  C_2p32/1 -> Mod_2p32/2  "two_p32"
  Shift_imu_dropout/1 -> OR_fault_inject/4  "imu_dropout_bit"
  Mod_2p32/1 -> DTC_t_us/1  "t_us_m"
  OR_fault_inject/1 -> RT_fault_inject/1  "fault_inject"
  RT_fault_inject/1 -> BC_in1k/5  "fault_inject"
  DTC_t_us/1 -> BC_in1k/3  "t_us"
  Sel_elec_hw/1 -> BC_in1k/2  "<di_word>"
  Sel_elec_hw/2 -> BC_in1k/4  "<reset_flag>"
  BC_in1k/1 -> in1k/1  "in1k"

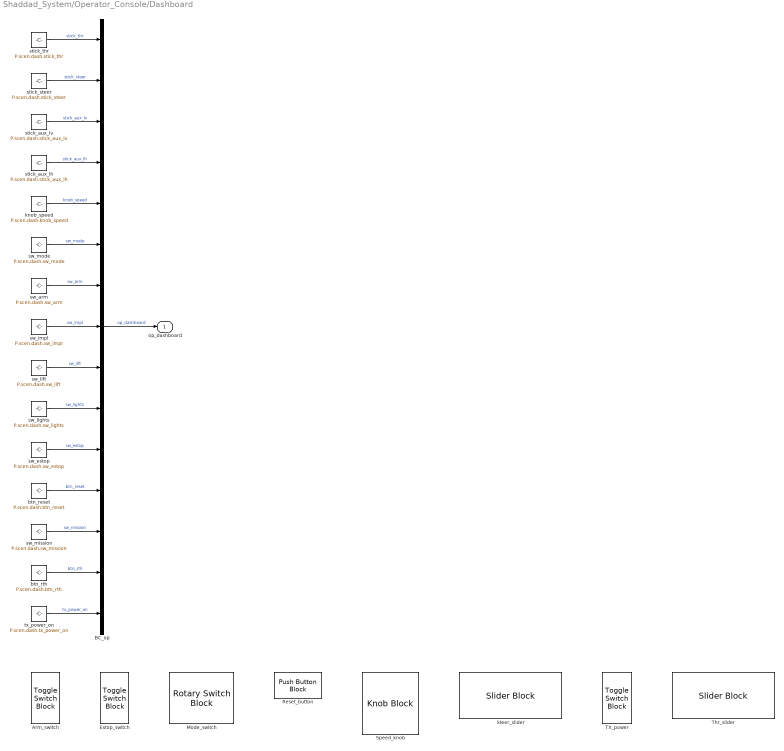
== system Shaddad_System/Operator_Console/Dashboard ==
  Arm_switch : ToggleSwitchBlock
  BC_op : BusCreator  Inputs=15  OutDataTypeStr=Bus: Bus_OperatorCmd  NonVirtualBus=on
  Estop_switch : ToggleSwitchBlock
  Mode_switch : RotarySwitchBlock
  Reset_button : PushButtonBlock  IconOnColor=[0.0, 0.39215686274509803, 0.0]  IconOffColor=[0.0, 1.0, 0.0]
  Speed_knob : KnobBlock  ScaleMin=-1  ScaleMax=1
  Steer_slider : SliderBlock  ScaleMin=-1  ScaleMax=1
  TX_power : ToggleSwitchBlock
  Thr_slider : SliderBlock  ScaleMin=-1  ScaleMax=1
  btn_reset : Constant  Value=P.scen.dash.btn_reset  OutDataTypeStr=double  SampleTime=Ts.scen
  btn_rth : Constant  Value=P.scen.dash.btn_rth  OutDataTypeStr=double  SampleTime=Ts.scen
  knob_speed : Constant  Value=P.scen.dash.knob_speed  OutDataTypeStr=double  SampleTime=Ts.scen
  stick_aux_lh : Constant  Value=P.scen.dash.stick_aux_lh  OutDataTypeStr=double  SampleTime=Ts.scen
  stick_aux_lv : Constant  Value=P.scen.dash.stick_aux_lv  OutDataTypeStr=double  SampleTime=Ts.scen
  stick_steer : Constant  Value=P.scen.dash.stick_steer  OutDataTypeStr=double  SampleTime=Ts.scen
  stick_thr : Constant  Value=P.scen.dash.stick_thr  OutDataTypeStr=double  SampleTime=Ts.scen
  sw_arm : Constant  Value=P.scen.dash.sw_arm  OutDataTypeStr=double  SampleTime=Ts.scen
  sw_estop : Constant  Value=P.scen.dash.sw_estop  OutDataTypeStr=double  SampleTime=Ts.scen
  sw_impl : Constant  Value=P.scen.dash.sw_impl  OutDataTypeStr=double  SampleTime=Ts.scen
  sw_lift : Constant  Value=P.scen.dash.sw_lift  OutDataTypeStr=double  SampleTime=Ts.scen
  sw_lights : Constant  Value=P.scen.dash.sw_lights  OutDataTypeStr=double  SampleTime=Ts.scen
  sw_mission : Constant  Value=P.scen.dash.sw_mission  OutDataTypeStr=double  SampleTime=Ts.scen
  sw_mode : Constant  Value=P.scen.dash.sw_mode  OutDataTypeStr=double  SampleTime=Ts.scen
  tx_power_on : Constant  Value=P.scen.dash.tx_power_on  OutDataTypeStr=double  SampleTime=Ts.scen
  op_dashboard : Outport  OutDataTypeStr=Bus: Bus_OperatorCmd
  wires:
  stick_thr/1 -> BC_op/1  "stick_thr"
  stick_steer/1 -> BC_op/2  "stick_steer"
  stick_aux_lv/1 -> BC_op/3  "stick_aux_lv"
  stick_aux_lh/1 -> BC_op/4  "stick_aux_lh"
  knob_speed/1 -> BC_op/5  "knob_speed"
  sw_mode/1 -> BC_op/6  "sw_mode"
  sw_arm/1 -> BC_op/7  "sw_arm"
  sw_impl/1 -> BC_op/8  "sw_impl"
  sw_lift/1 -> BC_op/9  "sw_lift"
  sw_lights/1 -> BC_op/10  "sw_lights"
  sw_estop/1 -> BC_op/11  "sw_estop"
  btn_reset/1 -> BC_op/12  "btn_reset"
  sw_mission/1 -> BC_op/13  "sw_mission"
  btn_rth/1 -> BC_op/14  "btn_rth"
  tx_power_on/1 -> BC_op/15  "tx_power_on"
  BC_op/1 -> op_dashboard/1  "op_dashboard"

== system Shaddad_System/Operator_Console/Joystick ==
  Joy_Map : MATLAB Function  TreatAsAtomicUnit=on  mask{m=P.scen.joy}
      mask prompts: m "Mapping (P.scen.joy)"
  Transmitter_USB : sl3dlib/Simulation 3D/Hardware Interface/Simulation 3D Joystick  joyid=1  adjustports=on  forcefeed=off
  op_joystick : Outport  OutDataTypeStr=Bus: Bus_OperatorCmd
  wires:
  Transmitter_USB/1 -> Joy_Map/1(axes)  "axes"
  Transmitter_USB/2 -> Joy_Map/2(buttons)  "buttons"
  Joy_Map/1(op) -> op_joystick/1  "op_joystick"

== system Shaddad_System/Operator_Console/RowDriver ==
  pose : Inport
  v_fwd : Inport  Port=2
  mcu_mode : Inport  Port=3
  tank_L : Inport  Port=4
  Driver : MATLAB Function  TreatAsAtomicUnit=on  mask{prm=P.scen.rowdrv}
      mask prompts: prm "Driver parameters (P.scen.rowdrv)"
  Ended : simulink/Logic and Bit Operations/Compare To Constant  relop=>  const=0.5  OutDataTypeStr=boolean
  Stop : Stop
  op_rowdriver : Outport  OutDataTypeStr=Bus: Bus_OperatorCmd
  wires:
  pose/1 -> Driver/1(pose)  "pose"
  v_fwd/1 -> Driver/2(v_fwd)  "v_fwd"
  mcu_mode/1 -> Driver/3(mcu_mode)  "mcu_mode"
  tank_L/1 -> Driver/4(tank_L)  "tank_L"
  Driver/1(op) -> op_rowdriver/1  "op_rowdriver"
  Driver/2(ended) -> Ended/1  "ended"
  Ended/1 -> Stop/1  "stop"

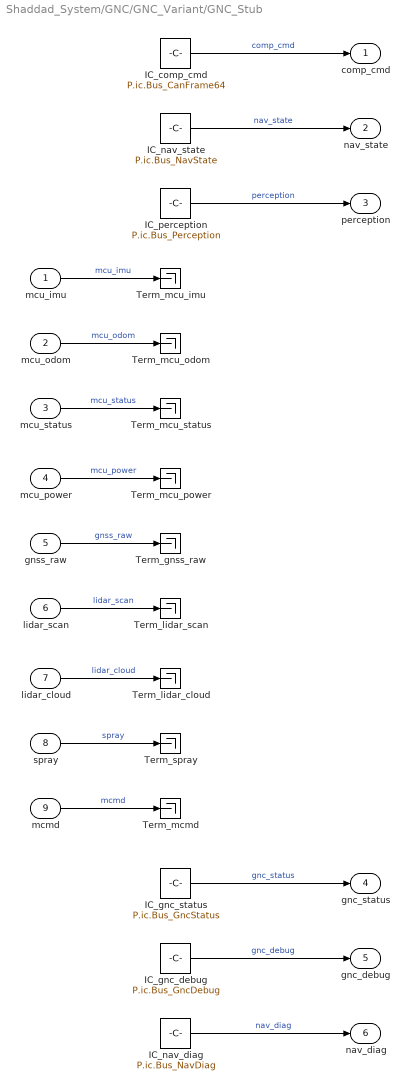
== system Shaddad_System/GNC/GNC_Variant/GNC_Stub ==
  mcu_imu : Inport  OutDataTypeStr=Bus: Bus_CanFrame64
  mcu_odom : Inport  Port=2  OutDataTypeStr=Bus: Bus_CanFrame64
  mcu_status : Inport  Port=3  OutDataTypeStr=Bus: Bus_CanFrame64
  mcu_power : Inport  Port=4  OutDataTypeStr=Bus: Bus_CanFrame64
  gnss_raw : Inport  Port=5  OutDataTypeStr=Bus: Bus_GnssRaw
  lidar_scan : Inport  Port=6  OutDataTypeStr=Bus: Bus_LidarScanRaw
  lidar_cloud : Inport  Port=7  OutDataTypeStr=Bus: Bus_LidarCloudRaw
  spray : Inport  Port=8  OutDataTypeStr=Bus: Bus_SprayDemand
  mcmd : Inport  Port=9  OutDataTypeStr=Bus: Bus_MissionCmd
  IC_comp_cmd : Constant  Value=P.ic.Bus_CanFrame64  OutDataTypeStr=Bus: Bus_CanFrame64  SampleTime=Ts.comm
  IC_gnc_debug : Constant  Value=P.ic.Bus_GncDebug  OutDataTypeStr=Bus: Bus_GncDebug  SampleTime=Ts.comm
  IC_gnc_status : Constant  Value=P.ic.Bus_GncStatus  OutDataTypeStr=Bus: Bus_GncStatus  SampleTime=Ts.gnc_status
  IC_nav_diag : Constant  Value=P.ic.Bus_NavDiag  OutDataTypeStr=Bus: Bus_NavDiag  SampleTime=Ts.ctrl
  IC_nav_state : Constant  Value=P.ic.Bus_NavState  OutDataTypeStr=Bus: Bus_NavState  SampleTime=Ts.ctrl
  IC_perception : Constant  Value=P.ic.Bus_Perception  OutDataTypeStr=Bus: Bus_Perception  SampleTime=Ts.hk
  Term_gnss_raw : Terminator
  Term_lidar_cloud : Terminator
  Term_lidar_scan : Terminator
  Term_mcmd : Terminator
  Term_mcu_imu : Terminator
  Term_mcu_odom : Terminator
  Term_mcu_power : Terminator
  Term_mcu_status : Terminator
  Term_spray : Terminator
  comp_cmd : Outport  OutDataTypeStr=Bus: Bus_CanFrame64
  nav_state : Outport  Port=2  OutDataTypeStr=Bus: Bus_NavState
  perception : Outport  Port=3  OutDataTypeStr=Bus: Bus_Perception
  gnc_status : Outport  Port=4  OutDataTypeStr=Bus: Bus_GncStatus
  gnc_debug : Outport  Port=5  OutDataTypeStr=Bus: Bus_GncDebug
  nav_diag : Outport  Port=6  OutDataTypeStr=Bus: Bus_NavDiag
  wires:
  mcu_imu/1 -> Term_mcu_imu/1  "mcu_imu"
  mcu_odom/1 -> Term_mcu_odom/1  "mcu_odom"
  mcu_status/1 -> Term_mcu_status/1  "mcu_status"
  mcu_power/1 -> Term_mcu_power/1  "mcu_power"
  gnss_raw/1 -> Term_gnss_raw/1  "gnss_raw"
  lidar_scan/1 -> Term_lidar_scan/1  "lidar_scan"
  lidar_cloud/1 -> Term_lidar_cloud/1  "lidar_cloud"
  spray/1 -> Term_spray/1  "spray"
  mcmd/1 -> Term_mcmd/1  "mcmd"
  IC_comp_cmd/1 -> comp_cmd/1  "comp_cmd"
  IC_nav_state/1 -> nav_state/1  "nav_state"
  IC_perception/1 -> perception/1  "perception"
  IC_gnc_status/1 -> gnc_status/1  "gnc_status"
  IC_gnc_debug/1 -> gnc_debug/1  "gnc_debug"
  IC_nav_diag/1 -> nav_diag/1  "nav_diag"

== matlab function Shaddad_System/Operator_Console/RowDriver/Driver ==
  settings: updateMethod=DISCRETE  sampleTime=Ts.scen  description=RC row test driver -> Bus_OperatorCmd, body utilities/row_driver_step.m (state utilities/row_driver_init.m), parameters P.scen.rowdrv (row_test_prm).
  data: pose input; op output Bus: Bus_OperatorCmd; v_fwd input; mcu_mode input; tank_L input; ended output; prm parameter
function [op, ended] = fcn(pose, v_fwd, mcu_mode, tank_L, prm)
%#codegen
% simulated RC row-test driver: what it sees -> Bus_OperatorCmd (utilities/row_driver_step.m, parameters
% P.scen.rowdrv); its state lives here (row_driver_init.m), its clock is t = k*Ts.scen from t = 0
persistent s
if isempty(s)
    s = row_driver_init(prm);
end
[op, s, ended] = row_driver_step(s, pose, v_fwd, mcu_mode, tank_L, prm);

== matlab function Shaddad_System/Operator_Console/Joystick/Joy_Map ==
  settings: updateMethod=DISCRETE  sampleTime=Ts.scen  description=Transmitter (USB joystick mode) -> Bus_OperatorCmd, body utilities/joy_map.m, mapping P.scen.joy.
  data: axes input; op output Bus: Bus_OperatorCmd; buttons input; m parameter
function op = fcn(axes, buttons, m)
%#codegen
% transmitter axes / buttons -> Bus_OperatorCmd (utilities/joy_map.m, mapping P.scen.joy)
op = joy_map(axes, buttons, m);
